simulink model "two_filter_comparision_model"  (R2025b)
settings: Solver=VariableStepAuto  StartTime=0.0  StopTime=0.5  RelTol=1e-3
values from neighbouring files (symbols this model uses):
  b_comp = b_comp(:).'    [two_filter_initialization.m]
  b_hb = b_hb(:).'    [two_filter_initialization.m]
undefined symbols (not defined in the file or in its folder): den, dspblkCoreblockFVToolHelper, gcbh, num
libraries: dspmlti4 x3, dspsrcs4 x1, dspfiltersrcs x1
settings Model: Creator=Prashant  LastModifiedBy=divijsharma
settings DataIOCC: SaveOutput=off  SignalLogging=off  DSMLogging=off  SaveTime=off  ReturnWorkspaceOutputs=off

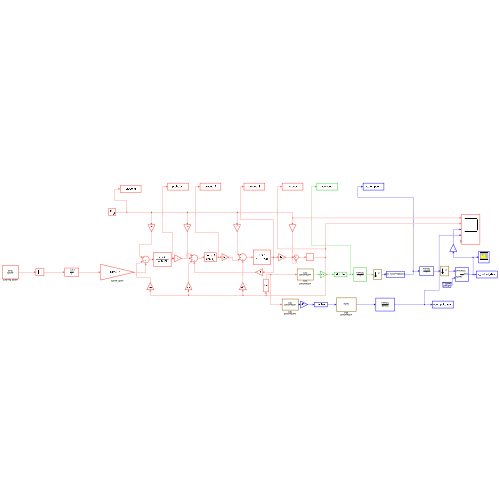
[thumbnail: Simulink's stored preview of the top-level diagram]
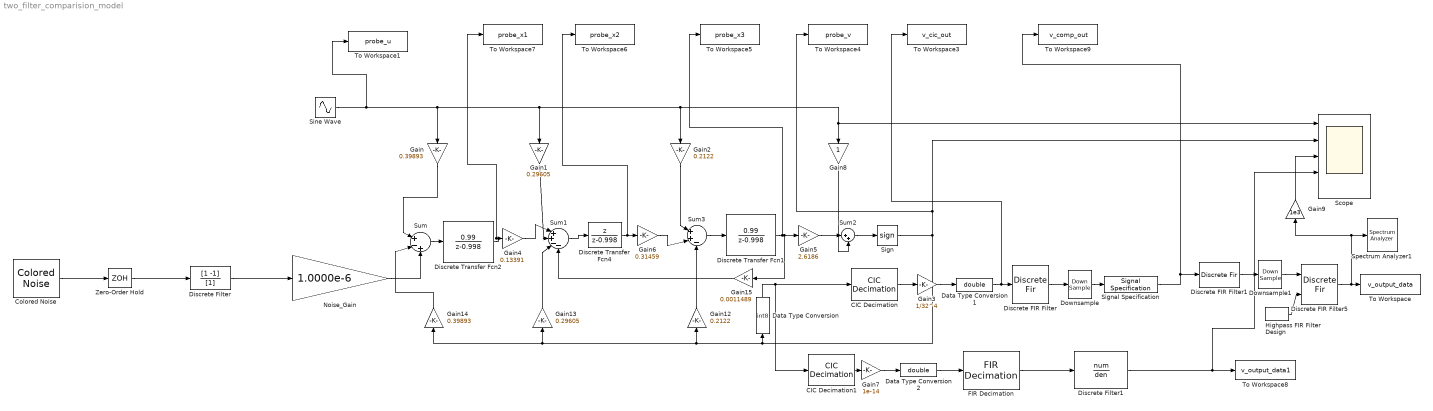
== system two_filter_comparision_model ==
  CIC Decimation : dspmlti4/CIC Decimation  filtFrom=Dialog parameters  filtobj=CICDECIM  ftype=Decimator  R=32  M=1  N=4  filterInternals=Full precision  BPS=[64 64 64 64]  FLPS=0  outputWordLength=32  outputFracLength=0  launchFVT=off  framing=Maintain input frame rate  RateOptions=Allow multirate processing
      settings: LibrarySourceBlock=|
      | dsphdlsupportfiltering/CIC
      | Decimation
  CIC Decimation1 : dspmlti4/CIC Decimation  filtFrom=Dialog parameters  filtobj=CICDECIM  ftype=Decimator  R=64  M=1  N=8  filterInternals=Full precision  BPS=[64 64 64 64]  FLPS=0  outputWordLength=32  outputFracLength=0  launchFVT=off  framing=Maintain input frame rate  RateOptions=Allow multirate processing
      settings: LibrarySourceBlock=|
      | dsphdlsupportfiltering/CIC
      | Decimation
  Colored Noise : dspsrcs4/Colored Noise  Color=pink  InverseFrequencyPower=1  BoundedOutput=off  NumChannels=1  OutputDataType=double  SamplesPerFrame=1  SampleTime=1/256000  RandomStream=mt19937ar with seed  Seed=67  SimulateUsing=Interpreted execution
  Data Type Conversion : DataTypeConversion  OutDataTypeStr=int8  RndMeth=Floor
  Data Type Conversion1 : DataTypeConversion  OutDataTypeStr=double  RndMeth=Floor
  Data Type Conversion2 : DataTypeConversion  OutDataTypeStr=double  RndMeth=Floor
  Discrete Transfer Fcn1 : DiscreteTransferFcn  LoadFcn=dspblkCoreblockFVToolHelper(gcbh,'load');  Numerator=[0.99]  Denominator=[1 -0.998]
      settings: CopyFcn=dspblkCoreblockFVToolHelper(gcbh,'copy');  DeleteFcn=dspblkCoreblockFVToolHelper(gcbh,'close');  ModelCloseFcn=dspblkCoreblockFVToolHelper(gcbh,'close');  PreSaveFcn=dspblkCoreblockFVToolHelper(gcbh,'presave');  PostSaveFcn=dspblkCoreblockFVToolHelper(gcbh,'postsave');  CloseFcn=dspblkCoreblockFVToolHelper(gcbh,'close');
  Discrete Transfer Fcn2 : DiscreteTransferFcn  LoadFcn=dspblkCoreblockFVToolHelper(gcbh,'load');  Numerator=[0.99]  Denominator=[1 -0.998]
      settings: CopyFcn=dspblkCoreblockFVToolHelper(gcbh,'copy');  DeleteFcn=dspblkCoreblockFVToolHelper(gcbh,'close');  ModelCloseFcn=dspblkCoreblockFVToolHelper(gcbh,'close');  PreSaveFcn=dspblkCoreblockFVToolHelper(gcbh,'presave');  PostSaveFcn=dspblkCoreblockFVToolHelper(gcbh,'postsave');  CloseFcn=dspblkCoreblockFVToolHelper(gcbh,'close');
  Discrete Transfer Fcn4 : DiscreteTransferFcn  LoadFcn=dspblkCoreblockFVToolHelper(gcbh,'load');  Numerator=[1 0]  Denominator=[1 -0.998]
      settings: CopyFcn=dspblkCoreblockFVToolHelper(gcbh,'copy');  DeleteFcn=dspblkCoreblockFVToolHelper(gcbh,'close');  ModelCloseFcn=dspblkCoreblockFVToolHelper(gcbh,'close');  PreSaveFcn=dspblkCoreblockFVToolHelper(gcbh,'presave');  PostSaveFcn=dspblkCoreblockFVToolHelper(gcbh,'postsave');  CloseFcn=dspblkCoreblockFVToolHelper(gcbh,'close');
  Discrete FIR Filter : DiscreteFir  LoadFcn=dspblkCoreblockFVToolHelper(gcbh,'load');  Coefficients=b_comp  InputProcessing=Columns as channels (frame based)
      settings: CopyFcn=dspblkCoreblockFVToolHelper(gcbh,'copy');  DeleteFcn=dspblkCoreblockFVToolHelper(gcbh,'close');  ModelCloseFcn=dspblkCoreblockFVToolHelper(gcbh,'close');  PreSaveFcn=dspblkCoreblockFVToolHelper(gcbh,'presave');  PostSaveFcn=dspblkCoreblockFVToolHelper(gcbh,'postsave');  CloseFcn=dspblkCoreblockFVToolHelper(gcbh,'close');
  Discrete FIR Filter1 : DiscreteFir  LoadFcn=dspblkCoreblockFVToolHelper(gcbh,'load');  FilterStructure=Direct form symmetric  Coefficients=b_hb  InputProcessing=Columns as channels (frame based)
      settings: CopyFcn=dspblkCoreblockFVToolHelper(gcbh,'copy');  DeleteFcn=dspblkCoreblockFVToolHelper(gcbh,'close');  ModelCloseFcn=dspblkCoreblockFVToolHelper(gcbh,'close');  PreSaveFcn=dspblkCoreblockFVToolHelper(gcbh,'presave');  PostSaveFcn=dspblkCoreblockFVToolHelper(gcbh,'postsave');  CloseFcn=dspblkCoreblockFVToolHelper(gcbh,'close');
  Discrete FIR Filter5 : DiscreteFir  LoadFcn=dspblkCoreblockFVToolHelper(gcbh,'load');  CoefSource=Input port
      settings: CopyFcn=dspblkCoreblockFVToolHelper(gcbh,'copy');  DeleteFcn=dspblkCoreblockFVToolHelper(gcbh,'close');  ModelCloseFcn=dspblkCoreblockFVToolHelper(gcbh,'close');  PreSaveFcn=dspblkCoreblockFVToolHelper(gcbh,'presave');  PostSaveFcn=dspblkCoreblockFVToolHelper(gcbh,'postsave');  CloseFcn=dspblkCoreblockFVToolHelper(gcbh,'close');  InputPortMap=u0,u1
  Discrete Filter : DiscreteFilter  LoadFcn=dspblkCoreblockFVToolHelper(gcbh,'load');  Numerator=[1 -1]  Denominator=[1]
      settings: CopyFcn=dspblkCoreblockFVToolHelper(gcbh,'copy');  DeleteFcn=dspblkCoreblockFVToolHelper(gcbh,'close');  ModelCloseFcn=dspblkCoreblockFVToolHelper(gcbh,'close');  PreSaveFcn=dspblkCoreblockFVToolHelper(gcbh,'presave');  PostSaveFcn=dspblkCoreblockFVToolHelper(gcbh,'postsave');  CloseFcn=dspblkCoreblockFVToolHelper(gcbh,'close');
  Discrete Filter1 : DiscreteFilter  LoadFcn=dspblkCoreblockFVToolHelper(gcbh,'load');  Numerator=num  Denominator=den
      settings: CopyFcn=dspblkCoreblockFVToolHelper(gcbh,'copy');  DeleteFcn=dspblkCoreblockFVToolHelper(gcbh,'close');  ModelCloseFcn=dspblkCoreblockFVToolHelper(gcbh,'close');  PreSaveFcn=dspblkCoreblockFVToolHelper(gcbh,'presave');  PostSaveFcn=dspblkCoreblockFVToolHelper(gcbh,'postsave');  CloseFcn=dspblkCoreblockFVToolHelper(gcbh,'close');
  Downsample : DownSample  RateOptions=Allow multirate processing  AllowArbitraryFixedInput=on
  Downsample1 : DownSample  RateOptions=Allow multirate processing  AllowArbitraryFixedInput=on
  FIR Decimation : dspmlti4/FIR Decimation  FilterSource=Dialog parameters  h=b_halfband  D=2  filtStruct=Direct form  FilterObject=FDECIM  framing=Allow multirate processing  AllowArbitraryInputLength=off  inputOffset=0  outputBufInitCond=0  roundingMode=Floor  overflowMode=off  firstCoeffDataTypeStr=Inherit: Same word length as input  firstCoeffMin=[]  firstCoeffMax=[]  firstCoeffLastDataTypeStr=Inherit: Same word length as input  outputDataTypeStr=Inherit: Same as accumulator  outputMin=[]  outputMax=[]  outputLastDataTypeStr=Inherit: Same as accumulator
      settings: LibrarySourceBlock=|
      | dsphdlsupportfiltering/FIR
      | Decimation
  Gain : Gain  Gain=0.39893
  Gain1 : Gain  Gain=0.29605
  Gain12 : Gain  Gain=0.2122
  Gain13 : Gain  Gain=0.29605
  Gain14 : Gain  Gain=0.39893
  Gain15 : Gain  Gain=0.0011489
  Gain2 : Gain  Gain=0.2122
  Gain3 : Gain  Gain=1/32^4  ParamDataTypeStr=double  OutDataTypeStr=double
  Gain4 : Gain  Gain=0.13391
  Gain5 : Gain  Gain=2.6186
  Gain6 : Gain  Gain=0.31459
  Gain7 : Gain  Gain=1e-14  ParamDataTypeStr=double  OutDataTypeStr=double
  Gain8 : Gain
  Gain9 : Gain  Gain=1e3  ParamDataTypeStr=double  OutDataTypeStr=double
  Highpass FIR Filter Design : dspfiltersrcs/Highpass FIR Filter Design  SmoothParameters=off  SmoothingFactor=0.6  FilterOrderPort=off  FilterOrder=128  MaxOrder=256  CutoffFrequencyPort=off  CutoffFrequency=1  Window=Hann  SidelobeAttenuationPort=off  SidelobeAttenuation=60  KaiserWindowParameterPort=off  KaiserWindowParameter=.5  OutputDataType=double  SampleTime=1/2e3  SimulateUsing=Interpreted execution
      settings: LibrarySourceBlock=dspfdesign/Highpass FIR Filter Design
  Noise_Gain : Gain  Gain=1.0000e-6
  Scope : Scope  NumInputPorts=5
      settings: ActiveDisplayYMinimum=-0.75  ActiveDisplayYMaximum=0.75
  Sign : Signum
  Signal Specification : SignalSpecification  Dimensions=[1 1]
  Sine Wave : Sin  Amplitude=0.6  Frequency=2*pi*100  Samples=500  SampleTime=1/256000
  Spectrum Analyzer1 : SpectrumAnalyzer  WindowPosition=[-128.000000,1.000000,1536.000000,741.000000,]  Visible=on  ScopeFrameLocation=window  WindowInvariantSamplesPerUpdate=on  Span=2000  StartFrequency=-1000  StopFrequency=1000  YLimits=[-369.8787 -296.0927]  SelectedToolstripTab=spectrumAnalyzerToolstrip.measurementsTab
  Sum : Sum  Inputs=|+-+
  Sum1 : Sum  Inputs=|++--
  Sum2 : Sum  Inputs=|++
  Sum3 : Sum  Inputs=|++-
  To Workspace : ToWorkspace  VariableName=v_output_data  SaveFormat=Timeseries  SampleTime=-1
  To Workspace1 : ToWorkspace  VariableName=probe_u  SaveFormat=Timeseries  SampleTime=-1
  To Workspace3 : ToWorkspace  VariableName=v_cic_out  SaveFormat=Timeseries  SampleTime=-1
  To Workspace4 : ToWorkspace  VariableName=probe_v  SaveFormat=Timeseries  SampleTime=-1
  To Workspace5 : ToWorkspace  VariableName=probe_x3  SaveFormat=Timeseries  SampleTime=-1
  To Workspace6 : ToWorkspace  VariableName=probe_x2  SaveFormat=Timeseries  SampleTime=-1
  To Workspace7 : ToWorkspace  VariableName=probe_x1  SaveFormat=Timeseries  SampleTime=-1
  To Workspace8 : ToWorkspace  VariableName=v_output_data1  SaveFormat=Timeseries  SampleTime=-1
  To Workspace9 : ToWorkspace  VariableName=v_comp_out  SaveFormat=Timeseries  SampleTime=-1
  Zero-Order Hold : ZeroOrderHold  SampleTime=1/256000
  wires:
  Sine Wave/1 -> To Workspace1/1, Gain8/1, Scope/1, Gain2/1, Gain1/1, Gain/1
  Gain3/1 -> Data Type Conversion1/1
  Colored Noise/1 -> Zero-Order Hold/1
  Discrete Filter/1 -> Noise_Gain/1
  Zero-Order Hold/1 -> Discrete Filter/1
  Sum2/1 -> Sign/1
  Gain2/1 -> Sum3/1
  Discrete Transfer Fcn1/1 -> To Workspace5/1, Gain15/1, Gain5/1
  Sum3/1 -> Discrete Transfer Fcn1/1
  Sign/1 -> Gain13/1, Gain14/1, Gain12/1, Data Type Conversion/1, To Workspace4/1, Scope/2
  CIC Decimation/1 -> Gain3/1
  Gain6/1 -> Sum3/2
  Gain15/1 -> Sum1/4
  Data Type Conversion1/1 -> To Workspace3/1, Discrete FIR Filter/1
  Sum1/1 -> Discrete Transfer Fcn4/1
  Discrete Transfer Fcn2/1 -> To Workspace7/1, Gain4/1
  Gain5/1 -> Sum2/1
  Noise_Gain/1 -> Sum/3
  Gain12/1 -> Sum3/3
  Discrete FIR Filter1/1 -> Downsample1/1
  Gain4/1 -> Sum1/1
  Sum/1 -> Discrete Transfer Fcn2/1
  Gain14/1 -> Sum/2
  Discrete Transfer Fcn4/1 -> To Workspace6/1, Gain6/1
  Data Type Conversion/1 -> CIC Decimation/1, CIC Decimation1/1
  Gain/1 -> Sum/1
  Gain1/1 -> Sum1/2
  Gain8/1 -> Sum2/2
  Gain13/1 -> Sum1/3
  Downsample1/1 -> Discrete FIR Filter5/1
  Downsample/1 -> Signal Specification/1
  Discrete FIR Filter/1 -> Downsample/1
  Signal Specification/1 -> To Workspace9/1, Discrete FIR Filter1/1
  FIR Decimation/1 -> Discrete Filter1/1
  Discrete Filter1/1 -> Scope/4, To Workspace8/1
  Gain7/1 -> Data Type Conversion2/1
  Data Type Conversion2/1 -> FIR Decimation/1
  CIC Decimation1/1 -> Gain7/1
  Gain9/1 -> Scope/3
  Discrete FIR Filter5/1 -> To Workspace/1, Gain9/1, Spectrum Analyzer1/1
  Highpass FIR Filter Design/1 -> Discrete FIR Filter5/2
